simulink library "ToyLib"  (R2023b)
settings: Solver=VariableStepAuto  StartTime=0.0  StopTime=10.0  RelTol=1e-3
settings Model: Creator=na  LastModifiedBy=na

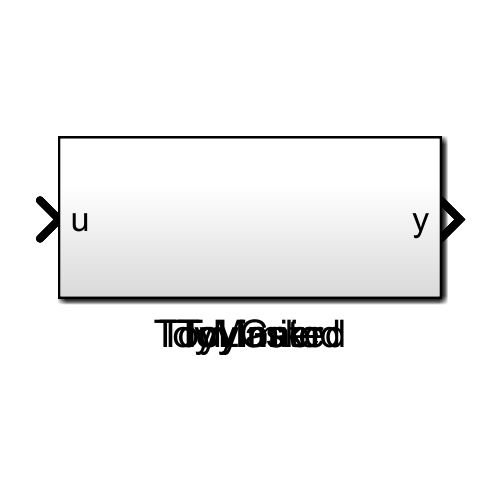
[thumbnail: Simulink's stored preview of the top-level diagram]
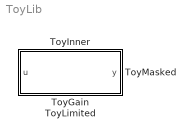
== system ToyLib ==
  ToyGain : Subsystem
  ToyInner : Subsystem
  ToyLimited : Subsystem  mask(signal){UpperLimit=1}
      mask prompts: UpperLimit "上限"
      mask help: 玩具限幅：输入乘增益后限幅
      mask Display: disp('玩具限幅');
  ToyMasked : Subsystem  mask(control){Kp=2}
      mask prompts: Kp "比例增益"
      mask help: 玩具掩码：Kp 增益 + Ki 备用
      mask Display: disp('玩具掩码');

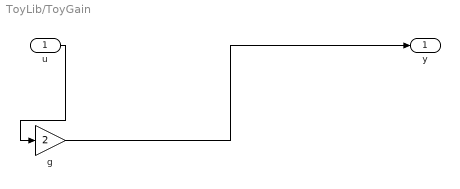
== system ToyLib/ToyGain ==
  u : Inport
  g : Gain  Gain=2
  y : Outport
  wires:
  u/1 -> g/1
  g/1 -> y/1

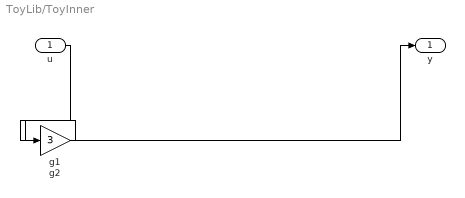
== system ToyLib/ToyInner ==
  u : Inport
  g1 : Gain  Gain=2
  g2 : Gain  Gain=3
  y : Outport
  wires:
  u/1 -> g1/1
  g1/1 -> g2/1
  g2/1 -> y/1

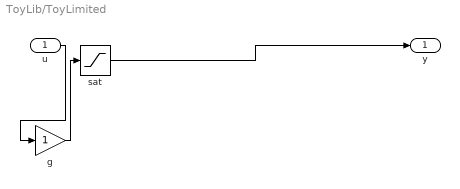
== system ToyLib/ToyLimited ==
  u : Inport
  g : Gain
  sat : Saturate
  y : Outport
  wires:
  u/1 -> g/1
  g/1 -> sat/1
  sat/1 -> y/1

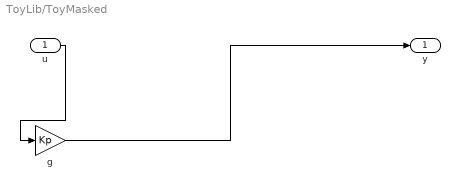
== system ToyLib/ToyMasked ==
  u : Inport
  g : Gain  Gain=Kp
  y : Outport
  wires:
  u/1 -> g/1
  g/1 -> y/1
